simulink model "Plant"  (R2018b)
settings: configuration reference "plant_config" (kept outside this file)
values from neighbouring files (symbols this model uses):
  ada =     [acdata.mat]    (also in aero_data.mat)
  ade =     [acdata.mat]    (also in aero_data.mat)
  adr =     [acdata.mat]    (also in aero_data.mat)
  adyn =     [acdata.mat]    (also in aero_data.mat)
  alat =     [acdata.mat]    (also in aero_data.mat)
  alon =     [acdata.mat]    (also in aero_data.mat)
  geo =     [acdata.mat]    (also in aero_data.mat)
  mc =     [acdata.mat]    (also in aero_data.mat)
  PLANT_EXPORT = Simulink.Parameter(PLANT_EXPORT_VALUE)    [plant_model_init.m]
undefined symbols (not defined in the file or in its folder): acc_x, acc_x_O, acc_y, acc_y_O, acc_z, acc_z_O, alt, alt_0, day, diff_pressure, DiscIntNeverNeededParam, fixType, flags, gSpeed, gyr_x, gyr_y, gyr_z, h_R, hAcc, heading, headingAcc, height, hMSL, hour, iTOW, lat, lon, M_BO, M_OB, mag_x, mag_y, mag_z, month, nano, numSV, pDOP, phi, PLANT_CONST, plant_model, pressure, psi, quat, reserved1, reserved2, rot_x_B, rot_y_B, rot_z_B, sAcc, sec, Sensor_Model, tAcc, temperature, temprature, theta, timestamp, Va, vAcc, valid, vel_x_O, vel_y_O ... (+7)
libraries: FMT_Model_Lib x22, simulink x13, dspsrcs4 x6, aerolibatmos2 x1
(part 2 of 3)

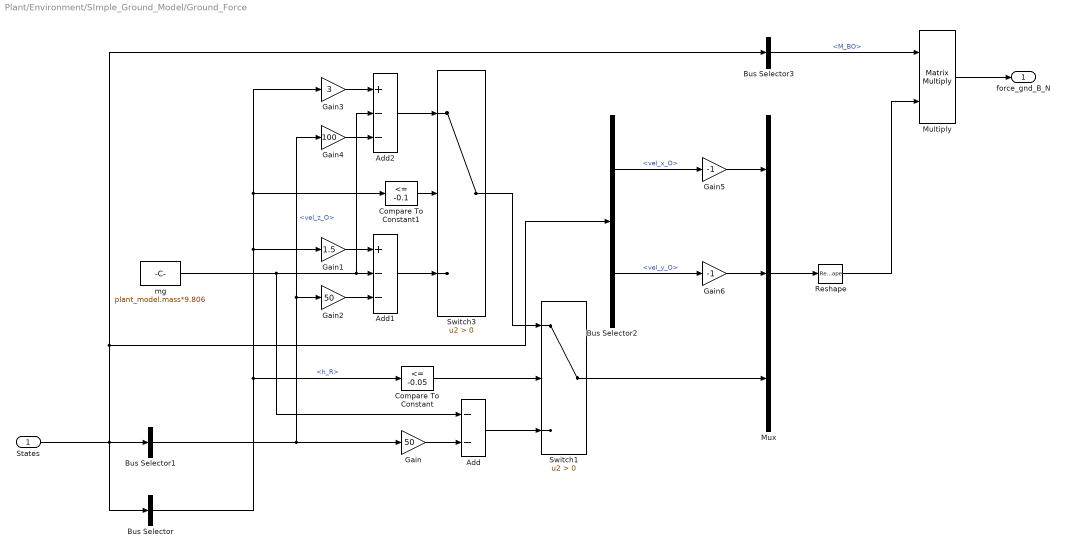
== system Plant/Environment/SImple_Ground_Model/Ground_Force ==
  States : Inport
  Add : Sum  Inputs=--
  Add1 : Sum  Inputs=+--
  Add2 : Sum  Inputs=+--
  Bus Selector : BusSelector  OutputSignals=Plant_States.h_R
  Bus Selector1 : BusSelector  OutputSignals=Plant_States.vel_z_O
  Bus Selector2 : BusSelector  OutputSignals=Plant_States.vel_x_O,Plant_States.vel_y_O
  Bus Selector3 : BusSelector  OutputSignals=Extended_States.M_BO
  Compare To Constant : simulink/Logic and Bit Operations/Compare To Constant  relop=<=  const=-0.05  OutDataTypeStr=boolean
  Compare To Constant1 : simulink/Logic and Bit Operations/Compare To Constant  relop=<=  const=-0.1  OutDataTypeStr=boolean
  Gain : Gain  Gain=50
  Gain1 : Gain  Gain=1.5
  Gain2 : Gain  Gain=50
  Gain3 : Gain  Gain=3
  Gain4 : Gain  Gain=100
  Gain5 : Gain  Gain=-1
  Gain6 : Gain  Gain=-1
  Multiply : Product  Multiplication=Matrix(*)
  Mux : Mux  Inputs=3
  Reshape : Reshape  OutputDimensionality=Customize  OutputDimensions=[3,1]
  Switch1 : Switch  Criteria=u2 > Threshold
  Switch3 : Switch  Criteria=u2 > Threshold
  mg : Constant  Value=plant_model.mass*9.806  OutDataTypeStr=single
  force_gnd_B_N : Outport
  wires:
  Switch1/1 -> Mux/3
  Bus Selector/1 -> Compare To Constant/1, Gain1/1, Gain3/1, Compare To Constant1/1  "<h_R>"
  Bus Selector1/1 -> Gain4/1, Gain2/1, Gain/1  "<vel_z_O>"
  Switch3/1 -> Switch1/1
  Gain1/1 -> Add1/1
  Gain5/1 -> Mux/1
  Gain3/1 -> Add2/1
  Compare To Constant/1 -> Switch1/2
  mg/1 -> Add/1, Add2/2, Add1/2
  Gain/1 -> Add/2
  Bus Selector2/2 -> Gain6/1  "<vel_y_O>"
  Gain2/1 -> Add1/3
  Add/1 -> Switch1/3
  Add2/1 -> Switch3/1
  Bus Selector2/1 -> Gain5/1  "<vel_x_O>"
  Gain6/1 -> Mux/2
  Compare To Constant1/1 -> Switch3/2
  Gain4/1 -> Add2/3
  Add1/1 -> Switch3/3
  Bus Selector3/1 -> Multiply/1  "<M_BO>"
  Mux/1 -> Reshape/1
  Multiply/1 -> force_gnd_B_N/1
  Reshape/1 -> Multiply/2
  States/1 -> Bus Selector/1, Bus Selector1/1, Bus Selector3/1, Bus Selector2/1

== system Plant/Environment/SImple_Ground_Model/Ground_Torque ==
  States : Inport
  Bus Selector2 : BusSelector  OutputSignals=Plant_States.rot_x_B,Plant_States.rot_y_B,Plant_States.rot_z_B
  Bus Selector3 : BusSelector  OutputSignals=Plant_States.phi,Plant_States.theta
  Constant : Constant  Value=0  OutDataTypeStr=single
  Gain1 : Gain  Gain=5
  Gain2 : Gain  Gain=plant_model.mass*9.806/30
  Gain3 : Gain  Gain=30
  Mux : Mux  Inputs=3
  Mux1 : Mux  Inputs=3
  Reshape1 : Reshape  OutputDimensionality=Customize  OutputDimensions=[3,1]
  Subtract : Sum  Inputs=--
  torque_gnd_B_Nm : Outport
  wires:
  Reshape1/1 -> Gain2/1
  States/1 -> Bus Selector3/1, Bus Selector2/1
  Subtract/1 -> Reshape1/1
  Bus Selector2/1 -> Mux1/1  "<rot_x_B>"
  Bus Selector2/2 -> Mux1/2  "<rot_y_B>"
  Bus Selector2/3 -> Mux1/3  "<rot_z_B>"
  Mux1/1 -> Gain1/1
  Gain1/1 -> Subtract/2
  Constant/1 -> Mux/3
  Mux/1 -> Gain3/1
  Gain2/1 -> torque_gnd_B_Nm/1
  Gain3/1 -> Subtract/1
  Bus Selector3/1 -> Mux/1  "<phi>"
  Bus Selector3/2 -> Mux/2  "<theta>"

== system Plant/Kinematic_Equation/Attitude_Dynamic/Quaternuin_Update ==
  omega_B_radPs : Inport
  reset : Inport  Port=2
  init_quat : Inport  Port=3
  Discrete-Time Integrator : DiscreteIntegrator  ExternalReset=level  InitialConditionSource=external  SampleTime=-1  ICPrevOutput=DiscIntNeverNeededParam  ICPrevScaledInput=DiscIntNeverNeededParam
  Gain : Gain  Gain=0.5  OutDataTypeStr=Inherit: Same as input
  Multiply : Product  Multiplication=Matrix(*)  OutDataTypeStr=Inherit: Same as first input
  Quaternion_Update_Maxtrix : Subsystem
  quat : Outport
  wires:
  Gain/1 -> Discrete-Time Integrator/1  "dot_q"
  Discrete-Time Integrator/1 -> quat/1, Multiply/2
  init_quat/1 -> Discrete-Time Integrator/3
  reset/1 -> Discrete-Time Integrator/2
  Multiply/1 -> Gain/1
  Quaternion_Update_Maxtrix/1(W) -> Multiply/1
  omega_B_radPs/1 -> Quaternion_Update_Maxtrix/1(omega_B_radPs)

== system Plant/Sensor_Model/Sensor_Airspeed/Airspeed ==
  Enable_Errors : Inport
  States : Inport  Port=2
  Bus Selector : BusSelector  OutputSignals=Extended_States.Va
  Gain : Gain  Gain=1.225/2
  Square : Math  Operator=square  SaturateOnIntegerOverflow=on
  Terminator : Terminator
  diff_pressure_Pa : Outport
  wires:
  States/1 -> Bus Selector/1
  Gain/1 -> diff_pressure_Pa/1
  Enable_Errors/1 -> Terminator/1
  Bus Selector/1 -> Square/1  "<Va>"
  Square/1 -> Gain/1

== system Plant/Sensor_Model/Sensor_Airspeed/Bus_Constructor ==
  diff_pressure_Pa : Inport  Unit=N/m^2
  timestamp_ms : Inport  Port=2
  Bus Assignment : BusAssignment  AssignedSignals=timestamp,diff_pressure
  Constant : Constant  Value=0  OutDataTypeStr=Bus: AirSpeed_Bus
  Data Type Conversion : DataTypeConversion  OutDataTypeStr=single
  Rate Transition : RateTransition  OutPortSampleTime=0.004
  Airspeed_Bus : Outport
  wires:
  Constant/1 -> Bus Assignment/1
  Data Type Conversion/1 -> Bus Assignment/3
  Bus Assignment/1 -> Rate Transition/1
  diff_pressure_Pa/1 -> Data Type Conversion/1
  Rate Transition/1 -> Airspeed_Bus/1
  timestamp_ms/1 -> Bus Assignment/2

== system Plant/Sensor_Model/Sensor_Barometer/Barometer ==
  Enable_Errors : Inport
  States : Inport  Port=2
  Physical_Model : Subsystem
  Sensor_Model : Subsystem
  pressure_Pa : Outport
  temprature_K : Outport  Port=2
  wires:
  Physical_Model/1(Pressure_Pa) -> Sensor_Model/2(u)
  Enable_Errors/1 -> Sensor_Model/1(Enable_Errors)
  States/1 -> Physical_Model/1(States)
  Sensor_Model/1(y) -> pressure_Pa/1
  Physical_Model/2(Temperature_K) -> temprature_K/1

== system Plant/Sensor_Model/Sensor_Barometer/Bus_Constructor ==
  pressure_Pa : Inport  Unit=N/m^2
  temperature_K : Inport  Port=2  Unit=K
  timestamp_ms : Inport  Port=3
  Bus Assignment : BusAssignment  AssignedSignals=timestamp,pressure,temperature
  Constant : Constant  Value=0  OutDataTypeStr=Bus: Barometer_Bus
  Constant2 : Constant  Value=273.15
  Data Type Conversion : DataTypeConversion  OutDataTypeStr=single
  Data Type Conversion1 : DataTypeConversion  OutDataTypeStr=single
  Rate Transition : RateTransition  OutPortSampleTime=0.01
  Sum1 : Sum  Inputs=|+-
  Barometer_Bus : Outport
  wires:
  Data Type Conversion1/1 -> Bus Assignment/4
  Constant/1 -> Bus Assignment/1
  Data Type Conversion/1 -> Bus Assignment/3
  Bus Assignment/1 -> Rate Transition/1
  pressure_Pa/1 -> Data Type Conversion/1
  temperature_K/1 -> Sum1/1
  Rate Transition/1 -> Barometer_Bus/1
  Sum1/1 -> Data Type Conversion1/1
  Constant2/1 -> Sum1/2
  timestamp_ms/1 -> Bus Assignment/2

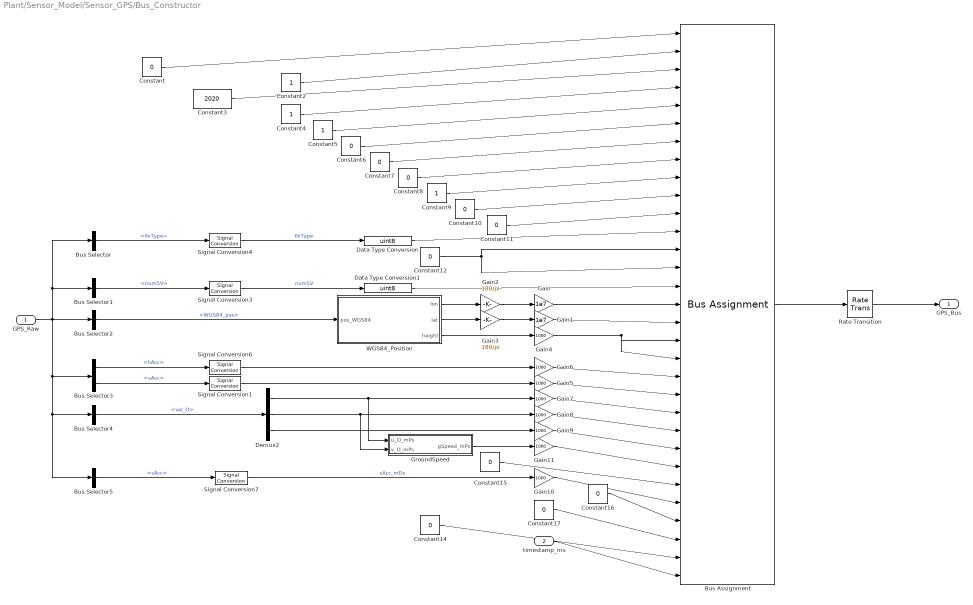
== system Plant/Sensor_Model/Sensor_GPS/Bus_Constructor ==
  GPS_Raw : Inport
  timestamp_ms : Inport  Port=2
  Bus Assignment : BusAssignment  AssignedSignals=iTOW,year,month,day,hour,min,sec,valid,tAcc,nano,fixType,flags,reserved1,numSV,lon,lat,height,hMSL,hAcc,vAcc,velN,velE,velD,gSpeed,heading,sAcc,headingAcc,pDOP,reserved2,timestamp
  Bus Selector : BusSelector  OutputSignals=fixType
  Bus Selector1 : BusSelector  OutputSignals=numSV
  Bus Selector2 : BusSelector  OutputSignals=WGS84_pos
  Bus Selector3 : BusSelector  OutputSignals=hAcc,vAcc
  Bus Selector4 : BusSelector  OutputSignals=vel_O
  Bus Selector5 : BusSelector  OutputSignals=sAcc
  Constant : Constant  Value=0  OutDataTypeStr=Bus: GPS_uBlox_Bus
  Constant10 : Constant  Value=0  OutDataTypeStr=uint32
  Constant11 : Constant  Value=0  OutDataTypeStr=int32
  Constant{6..8,12} (4 alike) : Constant  Value=0  OutDataTypeStr=uint8
  Constant14 : Constant  Value=0  OutDataTypeStr=uint16
  Constant15 : Constant  Value=0  OutDataTypeStr=int32
  Constant16 : Constant  Value=0  OutDataTypeStr=uint32
  Constant17 : Constant  Value=0  OutDataTypeStr=uint16
  Constant2 : Constant  OutDataTypeStr=uint32
  Constant3 : Constant  Value=2020  OutDataTypeStr=uint16
  Constant4 : Constant  OutDataTypeStr=uint8
  Constant5 : Constant  OutDataTypeStr=uint8
  Constant9 : Constant  OutDataTypeStr=uint8
  Data Type Conversion : DataTypeConversion  OutDataTypeStr=uint8
  Data Type Conversion1 : DataTypeConversion  OutDataTypeStr=uint8
  Demux2 : Demux  Outputs=3
  Gain : Gain  Gain=1e7  OutDataTypeStr=int32
      settings: AttributesFormatString=Gain: %<Gain>
  Gain1 : Gain  Gain=1e7  OutDataTypeStr=int32
      settings: AttributesFormatString=Gain: %<Gain>
  Gain10 : Gain  Gain=1000  OutDataTypeStr=uint32
      settings: AttributesFormatString=Gain: %<Gain>
  Gain{4,7..9,11} (5 alike) : Gain  Gain=1000  OutDataTypeStr=int32
      settings: AttributesFormatString=Gain: %<Gain>
  Gain2 : Gain  Gain=180/pi
      settings: AttributesFormatString=Gain: %<Gain>
  Gain3 : Gain  Gain=180/pi
      settings: AttributesFormatString=Gain: %<Gain>
  Gain5 : Gain  Gain=1000  OutDataTypeStr=uint32
      settings: AttributesFormatString=Gain: %<Gain>
  Gain6 : Gain  Gain=1000  OutDataTypeStr=uint32
      settings: AttributesFormatString=Gain: %<Gain>
  GroundSpeed : Subsystem
  Rate Transition : RateTransition  OutPortSampleTime=0.1
  Signal Conversion{1,3..4,6..7} (5 alike) : SignalConversion  OverrideOpt=off
  WGS84_Position : Subsystem
  GPS_Bus : Outport
  wires:
  Bus Selector5/1 -> Signal Conversion7/1  "<sAcc>"
  Bus Selector3/1 -> Signal Conversion6/1  "<hAcc>"
  Bus Selector1/1 -> Signal Conversion3/1  "<numSV>"
  Bus Selector4/1 -> Demux2/1  "<vel_O>"
  Gain5/1 -> Bus Assignment/21
  Constant15/1 -> Bus Assignment/26
  Data Type Conversion/1 -> Bus Assignment/12
  Constant17/1 -> Bus Assignment/29
  Gain4/1 -> Bus Assignment/19, Bus Assignment/18
  Constant16/1 -> Bus Assignment/28
  Gain3/1 -> Gain1/1
  Signal Conversion6/1 -> Gain6/1
  Gain6/1 -> Bus Assignment/20
  Gain11/1 -> Bus Assignment/25
  Gain8/1 -> Bus Assignment/23
  Gain7/1 -> Bus Assignment/22
  Gain10/1 -> Bus Assignment/27
  Constant/1 -> Bus Assignment/1
  Constant8/1 -> Bus Assignment/8
  Gain2/1 -> Gain/1
  Constant4/1 -> Bus Assignment/4
  Constant11/1 -> Bus Assignment/11
  Constant10/1 -> Bus Assignment/10
  Constant9/1 -> Bus Assignment/9
  Constant3/1 -> Bus Assignment/3
  Constant6/1 -> Bus Assignment/6
  Bus Assignment/1 -> Rate Transition/1
  Gain9/1 -> Bus Assignment/24
  Constant12/1 -> Bus Assignment/14, Bus Assignment/13
  Constant14/1 -> Bus Assignment/30
  GroundSpeed/1(gSpeed_mPs) -> Gain11/1
  Constant5/1 -> Bus Assignment/5
  Gain/1 -> Bus Assignment/16
  Data Type Conversion1/1 -> Bus Assignment/15
  Constant2/1 -> Bus Assignment/2
  Gain1/1 -> Bus Assignment/17
  Constant7/1 -> Bus Assignment/7
  Signal Conversion7/1 -> Gain10/1  "sAcc_mDs"
  Demux2/1 -> GroundSpeed/1(u_O_mPs), Gain7/1
  Demux2/2 -> Gain8/1, GroundSpeed/2(v_O_mPs)
  Demux2/3 -> Gain9/1
  Bus Selector2/1 -> WGS84_Position/1(pos_WGS84)  "<WGS84_pos>"
  WGS84_Position/1(lon) -> Gain2/1
  WGS84_Position/2(lat) -> Gain3/1
  WGS84_Position/3(height) -> Gain4/1
  Signal Conversion3/1 -> Data Type Conversion1/1  "numSV"
  Signal Conversion4/1 -> Data Type Conversion/1  "fixType"
  Bus Selector3/2 -> Signal Conversion1/1  "<vAcc>"
  Signal Conversion1/1 -> Gain5/1
  Rate Transition/1 -> GPS_Bus/1
  timestamp_ms/1 -> Bus Assignment/31
  GPS_Raw/1 -> Bus Selector3/1, Bus Selector4/1, Bus Selector5/1, Bus Selector2/1, Bus Selector1/1, Bus Selector/1
  Bus Selector/1 -> Signal Conversion4/1  "<fixType>"

== system Plant/Sensor_Model/Sensor_GPS/GPS ==
  Enable_Errors : Inport
  States : Inport  Port=2
  Bus_Constructor : Subsystem
  Physical_Model : Subsystem
  Sensor_Model : Subsystem
  GPS_Raw : Outport
  wires:
  Physical_Model/1(WGS84_pos_rad) -> Sensor_Model/2(WGS84_pos_rad)
  Physical_Model/2(vel_O_mPs) -> Sensor_Model/3(vel_O_mPs)
  States/1 -> Physical_Model/1(States)
  Enable_Errors/1 -> Sensor_Model/1(Enable_Errors)
  Sensor_Model/1(WGS84_pos_meas) -> Bus_Constructor/1(WGS84_pos_meas)
  Sensor_Model/2(vel_O_meas) -> Bus_Constructor/2(vel_O_meas)
  Sensor_Model/3(numSV) -> Bus_Constructor/3(numSV)
  Sensor_Model/4(fixType) -> Bus_Constructor/4(fixType)
  Sensor_Model/5(h_Acc_m) -> Bus_Constructor/5(h_Acc_m)
  Sensor_Model/6(v_Acc_m) -> Bus_Constructor/6(v_Acc_m)
  Sensor_Model/7(s_Acc_mDs) -> Bus_Constructor/7(s_Acc_mDs)
  Bus_Constructor/1(GPS_Raw) -> GPS_Raw/1

== system Plant/Sensor_Model/Sensor_IMU/Accelerometer ==
  States : Inport
  Enable_Errors : Inport  Port=2
  Bus_Constructor : Subsystem
  Physical_Model : Subsystem
  Sensor_Model : Subsystem
  Acc_Raw : Outport
  wires:
  Sensor_Model/1(y) -> Bus_Constructor/1(Output)
  States/1 -> Physical_Model/1(States)
  Physical_Model/1(sfor_B_mPs2) -> Sensor_Model/2(u)
  Bus_Constructor/1(Acc_Raw) -> Acc_Raw/1
  Enable_Errors/1 -> Physical_Model/2(Enable_Errors), Sensor_Model/1(Enable_Errors)

== system Plant/Sensor_Model/Sensor_IMU/Bus_Constructor ==
  Gyro_Raw : Inport
  Acc_Raw : Inport  Port=2
  timestamp_ms : Inport  Port=3
  Bus Assignment : BusAssignment  AssignedSignals=timestamp,gyr_x,gyr_y,gyr_z,acc_x,acc_y,acc_z
  Bus Selector : BusSelector  OutputSignals=Gyro_x_radPs,Gyro_y_radPs,Gyro_z_radPs
  Bus Selector1 : BusSelector  OutputSignals=Acc_x_mPs2,Acc_y_mPs2,Acc_z_mPs2
  Constant : Constant  Value=0  OutDataTypeStr=Bus: IMU_Bus
  IMU_Bus : Outport
  wires:
  Gyro_Raw/1 -> Bus Selector/1
  Acc_Raw/1 -> Bus Selector1/1
  Constant/1 -> Bus Assignment/1
  timestamp_ms/1 -> Bus Assignment/2
  Bus Assignment/1 -> IMU_Bus/1
  Bus Selector/1 -> Bus Assignment/3  "<Gyro_x_radPs>"
  Bus Selector/2 -> Bus Assignment/4  "<Gyro_y_radPs>"
  Bus Selector/3 -> Bus Assignment/5  "<Gyro_z_radPs>"
  Bus Selector1/1 -> Bus Assignment/6  "<Acc_x_mPs2>"
  Bus Selector1/2 -> Bus Assignment/7  "<Acc_y_mPs2>"
  Bus Selector1/3 -> Bus Assignment/8  "<Acc_z_mPs2>"

== system Plant/Sensor_Model/Sensor_IMU/Gyroscope ==
  States : Inport
  Enable_Errors : Inport  Port=2
  Bus_Constructor : Subsystem
  Physical_Model : Subsystem
  Sensor_Model : Subsystem
  Gyro_Raw : Outport
  wires:
  States/1 -> Physical_Model/1(States)
  Sensor_Model/1(y) -> Bus_Constructor/1(Output)
  Bus_Constructor/1(Gyro_Raw) -> Gyro_Raw/1
  Enable_Errors/1 -> Physical_Model/2(Enable_Errors), Sensor_Model/1(Enable_Errors)
  Physical_Model/1(gyr_B_radDs) -> Sensor_Model/2(u)

== system Plant/Sensor_Model/Sensor_MAG/Bus_Constructor ==
  Mag_Raw : Inport
  timestamp_ms : Inport  Port=2
  Bus Assignment : BusAssignment  AssignedSignals=timestamp,mag_x,mag_y,mag_z
  Bus Selector : BusSelector  OutputSignals=Mag_x_gauss,Mag_y_gauss,Mag_z_gauss
  Constant : Constant  Value=0  OutDataTypeStr=Bus: MAG_Bus
  Rate Transition : RateTransition  OutPortSampleTime=0.01
  MAG_Bus : Outport
  wires:
  Bus Assignment/1 -> Rate Transition/1
  Constant/1 -> Bus Assignment/1
  timestamp_ms/1 -> Bus Assignment/2
  Rate Transition/1 -> MAG_Bus/1
  Bus Selector/1 -> Bus Assignment/3  "<Mag_x_gauss>"
  Mag_Raw/1 -> Bus Selector/1
  Bus Selector/2 -> Bus Assignment/4  "<Mag_y_gauss>"
  Bus Selector/3 -> Bus Assignment/5  "<Mag_z_gauss>"

== system Plant/Sensor_Model/Sensor_MAG/Magnetometer ==
  States : Inport
  Enable_Errors : Inport  Port=2
  Bus_Constructor : Subsystem
  Physical_Model : Subsystem
  Sensor_Model : Subsystem
  Mag_Raw : Outport
  wires:
  Bus_Constructor/1(Mag_Raw) -> Mag_Raw/1
  Sensor_Model/1(y) -> Bus_Constructor/1(Output)
  States/1 -> Physical_Model/1(States)
  Physical_Model/1(mag_B_gauss) -> Sensor_Model/2(u)
  Enable_Errors/1 -> Sensor_Model/1(Enable_Errors)

== system Plant/Actuators/Aerodynamics Forces and Moments/Actuator Command/aileron_cmd ==
  actuator_cmd : Inport
  Bias : Bias  Bias=-1500
  Data Type Conversion : DataTypeConversion  OutDataTypeStr=single
  Gain2 : Gain  Gain=(30/500)*(pi/180)
  Selector : Selector  InputPortWidth=16  IndexOptions=Index vector (dialog)  Indices=6  OutputSizes=1
  aileron_cmd : Outport
  wires:
  actuator_cmd/1 -> Selector/1
  Gain2/1 -> aileron_cmd/1
  Bias/1 -> Gain2/1
  Selector/1 -> Data Type Conversion/1
  Data Type Conversion/1 -> Bias/1

== system Plant/Actuators/Aerodynamics Forces and Moments/Actuator Command/elevator_cmd ==
  actuator_cmd : Inport
  Bias : Bias  Bias=-1500
  Data Type Conversion : DataTypeConversion  OutDataTypeStr=single
  Gain2 : Gain  Gain=(30/500)*(pi/180)
  Selector : Selector  InputPortWidth=16  IndexOptions=Index vector (dialog)  Indices=8  OutputSizes=1
  elevator_cmd : Outport
  wires:
  Data Type Conversion/1 -> Bias/1
  Selector/1 -> Data Type Conversion/1
  Bias/1 -> Gain2/1
  Gain2/1 -> elevator_cmd/1
  actuator_cmd/1 -> Selector/1

== system Plant/Actuators/Aerodynamics Forces and Moments/Actuator Command/rudder_cmd ==
  actuator_cmd : Inport
  Bias : Bias  Bias=-1500
  Data Type Conversion : DataTypeConversion  OutDataTypeStr=single
  Gain2 : Gain  Gain=(30/500)*(pi/180)
  Selector : Selector  InputPortWidth=16  IndexOptions=Index vector (dialog)  Indices=9  OutputSizes=1
  rudder_cmd : Outport
  wires:
  Data Type Conversion/1 -> Bias/1
  Selector/1 -> Data Type Conversion/1
  Bias/1 -> Gain2/1
  Gain2/1 -> rudder_cmd/1
  actuator_cmd/1 -> Selector/1

== system Plant/Actuators/Aerodynamics Forces and Moments/Aerodynamic Coefficients/Actuator increments ==
  Incid : Inport
  ActData : Inport  Port=2
  Demux : Demux  Outputs=2
  Demux1 : Demux  Outputs=3
  Sum1 : Sum  Inputs=|+++
  Terminator : Terminator
  aileron : Subsystem
  elevator : Subsystem
  rudder : Subsystem
  Coeffs : Outport
  wires:
  Demux/2 -> Terminator/1
  Incid/1 -> Demux/1
  Demux/1 -> rudder/1(alpha), elevator/1(alpha), aileron/1(alpha)
  ActData/1 -> Demux1/1
  elevator/1(Coeffs) -> Sum1/2
  Sum1/1 -> Coeffs/1
  rudder/1(Coeffs) -> Sum1/3
  aileron/1(Coeffs) -> Sum1/1
  Demux1/3 -> rudder/2(dr)
  Demux1/2 -> elevator/2(de)
  Demux1/1 -> aileron/2(da)

== system Plant/Actuators/Aerodynamics Forces and Moments/Aerodynamic Coefficients/Basic Coefficients ==
  incid : Inport
  CD_basic : Lookup  InputValues=alon.alpha  Table=alon.CD
  CD_beta : Lookup2D  RowIndex=alat.beta  ColumnIndex=alat.alpha  Table=alat.CD
  CL_basic : Lookup  InputValues=alon.alpha  Table=alon.CL
  CL_beta : Lookup2D  RowIndex=alat.beta  ColumnIndex=alat.alpha  Table=alat.CL
  CY_basic : Lookup2D  RowIndex=alat.beta  ColumnIndex=alat.alpha  Table=alat.CY
  Cl_basic : Lookup2D  RowIndex=alat.beta  ColumnIndex=alat.alpha  Table=alat.Cl
  Cm_basic : Lookup  InputValues=alon.alpha  Table=alon.Cm
  Cm_beta : Lookup2D  RowIndex=alat.beta  ColumnIndex=alat.alpha  Table=alat.Cm
  Cn_basic : Lookup2D  RowIndex=alat.beta  ColumnIndex=alat.alpha  Table=alat.Cn  LookUpMeth=Interpolation-Use End Values
  Demux : Demux  Outputs=2
  Mux : Mux  Inputs=6
  Sum : Sum  Inputs=|++
  Sum1 : Sum  Inputs=|++
  Sum2 : Sum  Inputs=|++
  Coeffs : Outport
  wires:
  incid/1 -> Demux/1
  Demux/1 -> CY_basic/2, Cl_basic/2, Cm_basic/1, Cn_basic/2, CL_beta/2, CD_beta/2, Cm_beta/2, CL_basic/1, CD_basic/1
  CL_basic/1 -> Sum/1
  CD_basic/1 -> Sum1/1
  Cm_basic/1 -> Sum2/1
  Sum/1 -> Mux/2  "CL"
  Sum1/1 -> Mux/1  "CD"
  Sum2/1 -> Mux/5  "Cm"
  Mux/1 -> Coeffs/1
  CL_beta/1 -> Sum/2
  CD_beta/1 -> Sum1/2
  Cm_beta/1 -> Sum2/2
  CY_basic/1 -> Mux/3  "CY"
  Cl_basic/1 -> Mux/4  "Cl"
  Cn_basic/1 -> Mux/6  "Cn"
  Demux/2 -> CY_basic/1, Cl_basic/1, Cn_basic/1, CL_beta/1, CD_beta/1, Cm_beta/1

== system Plant/Actuators/Aerodynamics Forces and Moments/Aerodynamic Coefficients/Coeff_Decay ==
  u : Inport
  Va : Inport  Port=2
  Abs : Abs
  Constant : Constant  Value=10
  Divide : Product  Inputs=*/
  Multiply : Product
  Square : Math  Operator=square  SaturateOnIntegerOverflow=on
  Switch : Switch  Threshold=10
  y : Outport
  wires:
  Switch/1 -> y/1
  Divide/1 -> Square/1
  Constant/1 -> Divide/2
  u/1 -> Multiply/1, Switch/1
  Multiply/1 -> Switch/3  "dd1"
  Va/1 -> Abs/1
  Abs/1 -> Switch/2, Divide/1
  Square/1 -> Multiply/2

== system Plant/Actuators/Aerodynamics Forces and Moments/Aerodynamic Coefficients/body axis forces ==
  Incid : Inport
  Cl_DLY : Inport  Port=2
  Cl_xA : Fcn  Expr=-u[3]*cos(u[2])*cos(u[1])+u[4]*sin(u[1])
  Cl_yA : Fcn  Expr=-u[3]*sin(u[2])+u[5]
  Cl_zA : Fcn  Expr=-u[3]*cos(u[2])*sin(u[1])-u[4]*cos(u[1])
  Mux : Mux  Inputs=3
  Mux1 : Mux  Inputs=2
  Cl_XYZ : Outport
  wires:
  Mux/1 -> Cl_XYZ/1
  Cl_DLY/1 -> Mux1/2
  Incid/1 -> Mux1/1
  Cl_zA/1 -> Mux/3
  Cl_yA/1 -> Mux/2
  Cl_xA/1 -> Mux/1
  Mux1/1 -> Cl_zA/1, Cl_yA/1, Cl_xA/1

== system Plant/Actuators/Aerodynamics Forces and Moments/Aerodynamic Coefficients/body rate damping ==
  Incid : Inport
  pqr_n : Inport  Port=2
  Add : Sum  Inputs=+++
  Demux : Demux  Outputs=2
  Demux1 : Demux  Outputs=3
  Saturation : Saturate  UpperLimit=15/180*pi  LowerLimit=-15/180*pi
  Terminator : Terminator
  p : Subsystem
  p1 : Product  RndMeth=Zero
  q : Subsystem
  q1 : Product  RndMeth=Zero
  r : Subsystem
  r1 : Product  RndMeth=Zero
  Coeffs : Outport
  wires:
  Incid/1 -> Demux/1
  Demux/1 -> Saturation/1
  Demux/2 -> Terminator/1
  pqr_n/1 -> Demux1/1
  p/1(Coeffs) -> p1/1
  Demux1/1 -> p1/2
  q/1(Coeffs) -> q1/1
  r/1(Coeffs) -> r1/1
  Demux1/2 -> q1/2
  Demux1/3 -> r1/2
  q1/1 -> Add/2
  p1/1 -> Add/1
  r1/1 -> Add/3
  Add/1 -> Coeffs/1
  Saturation/1 -> p/1(alpha), q/1(alpha), r/1(alpha)

== system Plant/Actuators/Aerodynamics Forces and Moments/Aerodynamic Forces and Moments/Moments about CG due to Forces ==
  Forces : Inport
  CG : Inport  Port=2
  CP : Inport  Port=3
  Cross Product : FMT_Model_Lib/Math/Cross Product
      settings: SourceProductName=FMT Toolbox
  Sum : Sum  Inputs=|+-
  Moments : Outport
  wires:
  Cross Product/1 -> Moments/1
  Sum/1 -> Cross Product/2
  Forces/1 -> Cross Product/1
  CG/1 -> Sum/1
  CP/1 -> Sum/2

== system Plant/Actuators/MainMotor Forces and Moments/ESCs/Rotor_Delay ==
  in : Inport
  Discrete-Time Integrator : DiscreteIntegrator  gainval=K  SampleTime=-1  ICPrevOutput=DiscIntNeverNeededParam  ICPrevScaledInput=DiscIntNeverNeededParam
  Gain : Gain  Gain=1/T
  Subtract : Sum  Inputs=+-
  out : Outport
  wires:
  in/1 -> Subtract/1
  Subtract/1 -> Gain/1
  Gain/1 -> Discrete-Time Integrator/1
  Discrete-Time Integrator/1 -> Subtract/2, out/1

== system Plant/Actuators/MainMotor Forces and Moments/ESCs/Rotor_Speed ==
  u0 : Inport
  Add : Sum
  Compare To Constant : simulink/Logic and Bit Operations/Compare To Constant  relop=>  const=0.1  OutDataTypeStr=boolean
  Constant1 : Constant  Value=p  OutDataTypeStr=single
  Gain1 : Gain  Gain=k  OutDataTypeStr=Inherit: Same as input
  Multiply : Product
  Saturation1 : Saturate  UpperLimit=9999999  LowerLimit=0
  omega_B_radPs : Outport
  wires:
  Multiply/1 -> Saturation1/1
  Gain1/1 -> Add/1
  Saturation1/1 -> omega_B_radPs/1
  u0/1 -> Compare To Constant/1, Gain1/1
  Constant1/1 -> Add/2
  Compare To Constant/1 -> Multiply/1
  Add/1 -> Multiply/2

== system Plant/Actuators/MainMotor Forces and Moments/Force/Rotor_Thrust ==
  rotor_speed_radPs : Inport
  Multiply : Product  OutDataTypeStr=Inherit: Same as first input
  Square : Math  Operator=square  SaturateOnIntegerOverflow=on
  cT : Constant  Value=cT
  thrust_B_N : Outport
  wires:
  rotor_speed_radPs/1 -> Square/1
  Square/1 -> Multiply/1
  cT/1 -> Multiply/2
  Multiply/1 -> thrust_B_N/1

== system Plant/Actuators/Motors Forces and Moments/ESCs/Rotor_Delay ==
  in : Inport
  Discrete-Time Integrator : DiscreteIntegrator  gainval=K  SampleTime=-1  ICPrevOutput=DiscIntNeverNeededParam  ICPrevScaledInput=DiscIntNeverNeededParam
  Gain : Gain  Gain=1/T
  Subtract : Sum  Inputs=+-
  out : Outport
  wires:
  in/1 -> Subtract/1
  Subtract/1 -> Gain/1
  Gain/1 -> Discrete-Time Integrator/1
  Discrete-Time Integrator/1 -> Subtract/2, out/1

== system Plant/Actuators/Motors Forces and Moments/ESCs/Rotor_Speed ==
  u0 : Inport
  Add : Sum
  Compare To Constant : simulink/Logic and Bit Operations/Compare To Constant  relop=>  const=0.1  OutDataTypeStr=boolean
  Constant1 : Constant  Value=p  OutDataTypeStr=single
  Gain1 : Gain  Gain=k  OutDataTypeStr=Inherit: Same as input
  Multiply : Product
  Saturation1 : Saturate  UpperLimit=9999999  LowerLimit=0
  omega_B_radPs : Outport
  wires:
  Multiply/1 -> Saturation1/1
  Gain1/1 -> Add/1
  Saturation1/1 -> omega_B_radPs/1
  u0/1 -> Compare To Constant/1, Gain1/1
  Constant1/1 -> Add/2
  Compare To Constant/1 -> Multiply/1
  Add/1 -> Multiply/2

== system Plant/Actuators/Motors Forces and Moments/Force/Rotor_Thrust ==
  rotor_speed_radPs : Inport
  Multiply : Product  OutDataTypeStr=Inherit: Same as first input
  Square : Math  Operator=square  SaturateOnIntegerOverflow=on
  cT : Constant  Value=cT
  thrust_B_N : Outport
  wires:
  rotor_speed_radPs/1 -> Square/1
  Square/1 -> Multiply/1
  cT/1 -> Multiply/2
  Multiply/1 -> thrust_B_N/1

== system Plant/Actuators/Motors Forces and Moments/Torque/Gyroscopic_Torque ==
  rotor_speed_radPs : Inport
  omega_B_radPs : Inport  Port=2
  Add : Sum  Inputs=--++
  Constant : Constant  Value=[0;0;Im]  OutDataTypeStr=single
  Cross Product : FMT_Model_Lib/Math/Cross Product
      settings: SourceProductName=FMT Toolbox
  Demux : Demux
  Multiply : Product
  gyroscopic_torque : Outport
  wires:
  Demux/1 -> Add/1
  Constant/1 -> Cross Product/1
  Demux/4 -> Add/4
  Add/1 -> Multiply/1
  Demux/3 -> Add/3
  Demux/2 -> Add/2
  omega_B_radPs/1 -> Multiply/2
  Multiply/1 -> Cross Product/2
  Cross Product/1 -> gyroscopic_torque/1
  rotor_speed_radPs/1 -> Demux/1

== system Plant/Actuators/Motors Forces and Moments/Torque/Rotor_Torque ==
  rotor_speed_radPs : Inport
  Multiply : Product  Multiplication=Matrix(*)
  Square : Math  Operator=square  SaturateOnIntegerOverflow=on
  X_Frame_CM : Constant  Value=[-L*cT,L*cT,L*cT,-L*cT;L*cT,-L*cT,L*cT,-L*cT;cQ,cQ,-cQ,-cQ]  OutDataTypeStr=single
  rotor_torque : Outport
  wires:
  X_Frame_CM/1 -> Multiply/1
  Square/1 -> Multiply/2
  Multiply/1 -> rotor_torque/1
  rotor_speed_radPs/1 -> Square/1

== system Plant/Kinematic_Equation/Attitude_Dynamic/Quaternuin_Update/Quaternion_Update_Maxtrix ==
  omega_B_radPs : Inport
  Constant{,1..3} (4 alike) : Constant  Value=0  OutDataTypeStr=single
  Demux : Demux  Outputs=3
  Gain{1..4,6..7} (6 alike) : Gain  Gain=-1  OutDataTypeStr=Inherit: Same as input
  Matrix Concatenate{,1..3} (4 alike) : Concatenate  NumInputs=4
  Matrix Concatenate4 : Concatenate  NumInputs=4  Mode=Multidimensional array  ConcatenateDimension=2
  W : Outport
  wires:
  Gain1/1 -> Matrix Concatenate1/1
  Gain7/1 -> Matrix Concatenate3/2
  Matrix Concatenate2/1 -> Matrix Concatenate4/3  "col3"
  Constant2/1 -> Matrix Concatenate2/3
  Matrix Concatenate4/1 -> W/1
  Demux/1 -> Matrix Concatenate/2, Gain1/1, Gain4/1, Matrix Concatenate3/3  "w1"
  Matrix Concatenate/1 -> Matrix Concatenate4/1  "col1"
  Matrix Concatenate1/1 -> Matrix Concatenate4/2  "col2"
  Constant3/1 -> Matrix Concatenate3/4
  Gain6/1 -> Matrix Concatenate3/1
  Constant1/1 -> Matrix Concatenate1/2
  Matrix Concatenate3/1 -> Matrix Concatenate4/4  "col4"
  Demux/2 -> Matrix Concatenate1/4, Gain3/1, Gain7/1, Matrix Concatenate/3  "w2"
  Constant/1 -> Matrix Concatenate/1
  Gain3/1 -> Matrix Concatenate2/1
  Demux/3 -> Gain2/1, Matrix Concatenate2/2, Gain6/1, Matrix Concatenate/4  "w3"
  Gain2/1 -> Matrix Concatenate1/3
  omega_B_radPs/1 -> Demux/1
  Gain4/1 -> Matrix Concatenate2/4

== system Plant/Sensor_Model/Sensor_Barometer/Barometer/Physical_Model ==
  States : Inport
  Bus Selector1 : BusSelector  OutputSignals=Plant_States.alt
  Data Type Conversion : DataTypeConversion  OutDataTypeStr=single
  ISA Atmosphere Model : aerolibatmos2/ISA Atmosphere Model  custom=off  g=9.80665  gamma=1.4  R=287.0531  L=0.0065  h_trop=11000  h_strat=20000  rho0=1.225  P0=101325  T0=288.15  h0=0
      settings: SourceProductName=Aerospace Blockset
  Terminator : Terminator
  Terminator1 : Terminator
  Pressure_Pa : Outport
  Temperature_K : Outport  Port=2
  wires:
  States/1 -> Bus Selector1/1
  ISA Atmosphere Model/1 -> Temperature_K/1
  ISA Atmosphere Model/2 -> Terminator1/1
  ISA Atmosphere Model/4 -> Terminator/1
  Bus Selector1/1 -> Data Type Conversion/1  "<alt>"
  ISA Atmosphere Model/3 -> Pressure_Pa/1
  Data Type Conversion/1 -> ISA Atmosphere Model/1

== system Plant/Sensor_Model/Sensor_Barometer/Barometer/Sensor_Model ==
  Enable_Errors : Inport
  u : Inport  Port=2
  Add : Sum  InputSameDT=on  OutDataTypeStr=Inherit: Same as first input
  Saturation : Saturate  UpperLimit=Sensor_Model.Baro.Upper_limit  LowerLimit=Sensor_Model.Baro.Lower_limit  OutDataTypeStr=single
  Sensor_Error : Subsystem
  Sensor_Noise : Subsystem
  Switch : Switch  Criteria=u2 > Threshold
  y : Outport
  wires:
  Switch/1 -> y/1
  Saturation/1 -> Add/1
  Sensor_Error/1(y) -> Saturation/1
  Enable_Errors/1 -> Switch/2
  u/1 -> Switch/3, Sensor_Error/1(u)
  Add/1 -> Switch/1
  Sensor_Noise/1(noise) -> Add/2

== system Plant/Sensor_Model/Sensor_GPS/Bus_Constructor/GroundSpeed ==
  u_O_mPs : Inport
  v_O_mPs : Inport  Port=2
  Add : Sum
  Math Function : Math  Operator=square  SaturateOnIntegerOverflow=on
  Math Function1 : Math  Operator=square  SaturateOnIntegerOverflow=on
  Saturation : Saturate  UpperLimit=inf  LowerLimit=0
  Sqrt : Sqrt  SaturateOnIntegerOverflow=on
  gSpeed_mPs : Outport
  wires:
  Sqrt/1 -> gSpeed_mPs/1
  Math Function/1 -> Add/1
  Math Function1/1 -> Add/2
  Saturation/1 -> Sqrt/1
  Add/1 -> Saturation/1
  u_O_mPs/1 -> Math Function/1
  v_O_mPs/1 -> Math Function1/1

== system Plant/Sensor_Model/Sensor_GPS/Bus_Constructor/WGS84_Position ==
  pos_WGS84 : Inport
  Demux1 : Demux  Outputs=3
  Signal Conversion : SignalConversion  OverrideOpt=off
  Signal Conversion1 : SignalConversion  OverrideOpt=off
  Signal Conversion2 : SignalConversion  OverrideOpt=off
  lon : Outport
  lat : Outport  Port=2
  height : Outport  Port=3
  wires:
  Demux1/3 -> Signal Conversion2/1  "POS_h_WGS84"
  Signal Conversion/1 -> lon/1
  Demux1/1 -> Signal Conversion/1  "POS_lon_WGS84"
  pos_WGS84/1 -> Demux1/1
  Demux1/2 -> Signal Conversion1/1  "POS_lat_WGS84"
  Signal Conversion1/1 -> lat/1
  Signal Conversion2/1 -> height/1

== system Plant/Sensor_Model/Sensor_GPS/GPS/Bus_Constructor ==
  WGS84_pos_meas : Inport
  vel_O_meas : Inport  Port=2
  numSV : Inport  Port=3
  fixType : Inport  Port=4
  h_Acc_m : Inport  Port=5
  v_Acc_m : Inport  Port=6
  s_Acc_mDs : Inport  Port=7
  Bus Creator : BusCreator  Inputs=7
  GPS_Raw : Outport
  wires:
  WGS84_pos_meas/1 -> Bus Creator/1  "WGS84_pos"
  vel_O_meas/1 -> Bus Creator/2  "vel_O"
  numSV/1 -> Bus Creator/3  "numSV"
  fixType/1 -> Bus Creator/4  "fixType"
  h_Acc_m/1 -> Bus Creator/5  "hAcc"
  v_Acc_m/1 -> Bus Creator/6  "vAcc"
  s_Acc_mDs/1 -> Bus Creator/7  "sAcc"
  Bus Creator/1 -> GPS_Raw/1

== system Plant/Sensor_Model/Sensor_GPS/GPS/Physical_Model ==
  note: Transfer Delay
  States : Inport
  Bus Selector : BusSelector  OutputSignals=Plant_States.lon,Plant_States.lat,Plant_States.alt
  Bus Selector1 : BusSelector  OutputSignals=Plant_States.vel_x_O,Plant_States.vel_y_O,Plant_States.vel_z_O
  Delay : Delay  DelayLength=150/(PLANT_CONST.dt*1e3)
  Delay1 : Delay  DelayLength=100/(PLANT_CONST.dt*1e3)
  Vector Concatenate : Concatenate  NumInputs=3  Mode=Multidimensional array
  Vector Concatenate1 : Concatenate  NumInputs=3  Mode=Multidimensional array
  WGS84_pos_rad : Outport  Unit=rad/s
  vel_O_mPs : Outport  Port=2  Unit=m/s  PortDimensions=[3 1]
  wires:
  Bus Selector/3 -> Vector Concatenate/3  "<alt>"
  Bus Selector/2 -> Vector Concatenate/2  "<lat>"
  Bus Selector/1 -> Vector Concatenate/1  "<lon>"
  Vector Concatenate/1 -> Delay/1
  Bus Selector1/2 -> Vector Concatenate1/2  "<vel_y_O>"
  Bus Selector1/3 -> Vector Concatenate1/3  "<vel_z_O>"
  States/1 -> Bus Selector1/1, Bus Selector/1
  Vector Concatenate1/1 -> Delay1/1
  Bus Selector1/1 -> Vector Concatenate1/1  "<vel_x_O>"
  Delay/1 -> WGS84_pos_rad/1
  Delay1/1 -> vel_O_mPs/1

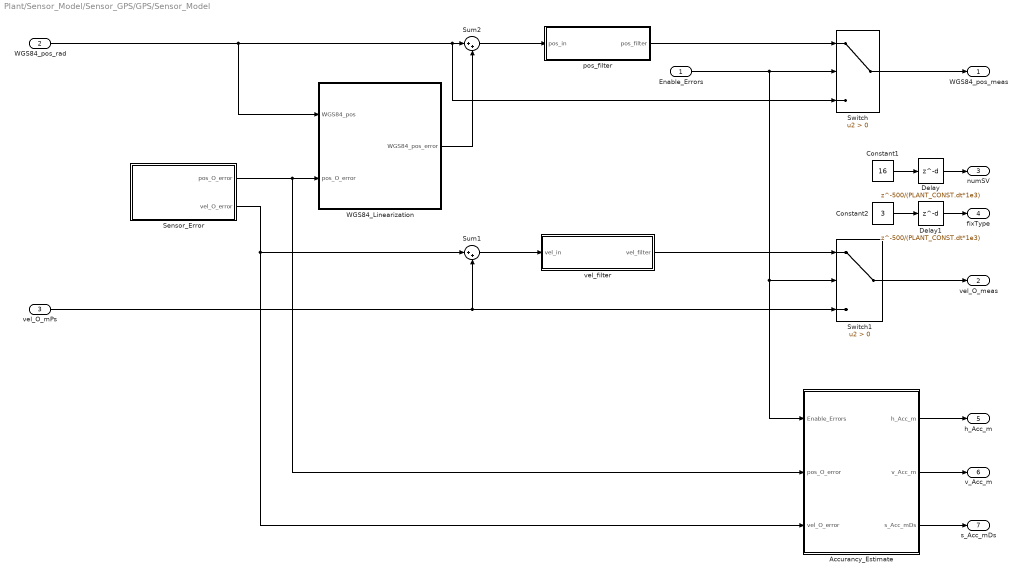
== system Plant/Sensor_Model/Sensor_GPS/GPS/Sensor_Model ==
  Enable_Errors : Inport
  WGS84_pos_rad : Inport  Port=2
  vel_O_mPs : Inport  Port=3
  Accurancy_Estimate : Subsystem
  Constant1 : Constant  Value=16  OutDataTypeStr=Inherit: Inherit via back propagation
  Constant2 : Constant  Value=3  OutDataTypeStr=Inherit: Inherit via back propagation
  Delay : Delay  DelayLength=500/(PLANT_CONST.dt*1e3)
  Delay1 : Delay  DelayLength=500/(PLANT_CONST.dt*1e3)
  Sensor_Error : Subsystem
  Sum1 : Sum  Inputs=|++
  Sum2 : Sum  Inputs=|++
  Switch : Switch  Criteria=u2 > Threshold
  Switch1 : Switch  Criteria=u2 > Threshold
  WGS84_Linearization : Subsystem
  pos_filter : Subsystem
  vel_filter : Subsystem
  WGS84_pos_meas : Outport
  vel_O_meas : Outport  Port=2
  numSV : Outport  Port=3
  fixType : Outport  Port=4
  h_Acc_m : Outport  Port=5
  v_Acc_m : Outport  Port=6
  s_Acc_mDs : Outport  Port=7
  wires:
  Constant2/1 -> Delay1/1
  Constant1/1 -> Delay/1
  Switch/1 -> WGS84_pos_meas/1
  Switch1/1 -> vel_O_meas/1
  Sum2/1 -> pos_filter/1(pos_in)
  Sensor_Error/1(pos_O_error) -> Accurancy_Estimate/2(pos_O_error), WGS84_Linearization/2(pos_O_error)
  Sum1/1 -> vel_filter/1(vel_in)
  Sensor_Error/2(vel_O_error) -> Accurancy_Estimate/3(vel_O_error), Sum1/1
  WGS84_Linearization/1(WGS84_pos_error) -> Sum2/2
  Accurancy_Estimate/1(h_Acc_m) -> h_Acc_m/1
  Accurancy_Estimate/3(s_Acc_mDs) -> s_Acc_mDs/1
  Accurancy_Estimate/2(v_Acc_m) -> v_Acc_m/1
  pos_filter/1(pos_filter) -> Switch/1
  WGS84_pos_rad/1 -> Switch/3, Sum2/1, WGS84_Linearization/1(WGS84_pos)
  vel_O_mPs/1 -> Switch1/3, Sum1/2
  vel_filter/1(vel_filter) -> Switch1/1
  Enable_Errors/1 -> Switch/2, Accurancy_Estimate/1(Enable_Errors), Switch1/2
  Delay/1 -> numSV/1
  Delay1/1 -> fixType/1

== system Plant/Sensor_Model/Sensor_IMU/Accelerometer/Bus_Constructor ==
  Output : Inport
  Bus Creator : BusCreator  Inputs=3
  Demux : Demux  Outputs=3
  Acc_Raw : Outport
  wires:
  Demux/2 -> Bus Creator/2  "Acc_y_mPs2"
  Demux/3 -> Bus Creator/3  "Acc_z_mPs2"
  Demux/1 -> Bus Creator/1  "Acc_x_mPs2"
  Bus Creator/1 -> Acc_Raw/1
  Output/1 -> Demux/1

== system Plant/Sensor_Model/Sensor_IMU/Accelerometer/Physical_Model ==
  States : Inport
  Enable_Errors : Inport  Port=2
  Sum : Sum  Inputs=|++
  Switch : Switch  Criteria=u2 > Threshold  OutDataTypeStr=single
  Vibration_Model : Subsystem  TreatAsAtomicUnit=on  mask{gain=Sensor_Model.Acc.Vibration.Gain}
      mask prompts: gain "Vibration gain"
      mask help: propeller vibration model
      settings: RTWSystemCode=Inline
  prop_vel : Subsystem
  specific_force : Subsystem
  sfor_B_mPs2 : Outport  Unit=m/s^2
  wires:
  States/1 -> specific_force/1(States), prop_vel/1(States)
  Switch/1 -> sfor_B_mPs2/1
  prop_vel/1(omega_radDs) -> Vibration_Model/1(prop_rot_radPs)
  specific_force/1(sfor_B_mPs2) -> Sum/2, Switch/3
  Enable_Errors/1 -> Switch/2
  Vibration_Model/1(vibration) -> Sum/1
  Sum/1 -> Switch/1

== system Plant/Sensor_Model/Sensor_IMU/Accelerometer/Sensor_Model ==
  Enable_Errors : Inport
  u : Inport  Port=2
  First Order LPF : FMT_Model_Lib/Filter/First Order LPF  fc=Sensor_Model.Acc.Cutoff_frequency_Hz
      settings: SourceProductName=FMT Toolbox
  Saturation : Saturate  UpperLimit=Sensor_Model.Acc.Upper_limit  LowerLimit=Sensor_Model.Acc.Lower_limit
  Sensor_Error : Subsystem
  Sensor_Noise : Subsystem
  Sum : Sum  Inputs=|++
  Switch : Switch  Criteria=u2 > Threshold
  y : Outport
  wires:
  Switch/1 -> y/1
  Saturation/1 -> Sum/1
  First Order LPF/1 -> Saturation/1
  Sensor_Error/1(y) -> First Order LPF/1
  Sensor_Noise/1(noise) -> Sum/2
  Enable_Errors/1 -> Switch/2
  u/1 -> Switch/3, Sensor_Error/1(u)
  Sum/1 -> Switch/1

== system Plant/Sensor_Model/Sensor_IMU/Gyroscope/Bus_Constructor ==
  Output : Inport
  Bus Creator : BusCreator  Inputs=3
  Demux : Demux  Outputs=3
  Gyro_Raw : Outport
  wires:
  Demux/1 -> Bus Creator/1  "Gyro_x_radPs"
  Demux/2 -> Bus Creator/2  "Gyro_y_radPs"
  Demux/3 -> Bus Creator/3  "Gyro_z_radPs"
  Bus Creator/1 -> Gyro_Raw/1
  Output/1 -> Demux/1

== system Plant/Sensor_Model/Sensor_IMU/Gyroscope/Physical_Model ==
  States : Inport
  Enable_Errors : Inport  Port=2
  Sum : Sum  Inputs=|++
  Switch : Switch  Criteria=u2 > Threshold
  Vibration_Model : Subsystem  TreatAsAtomicUnit=on  mask{gain=Sensor_Model.Gyro.Vibration.Gain}
      mask prompts: gain "Vibration gain"
      mask help: propeller vibration model
      settings: RTWSystemCode=Inline
  prop_vel : Subsystem
  rotation_speed : Subsystem
  gyr_B_radDs : Outport  Unit=rad/s
  wires:
  States/1 -> rotation_speed/1(States), prop_vel/1(States)
  Switch/1 -> gyr_B_radDs/1
  prop_vel/1(omega_radPs) -> Vibration_Model/1(prop_rot_radPs)
  rotation_speed/1(rot_radPs) -> Sum/2, Switch/3
  Enable_Errors/1 -> Switch/2
  Vibration_Model/1(vibration) -> Sum/1
  Sum/1 -> Switch/1

== system Plant/Sensor_Model/Sensor_IMU/Gyroscope/Sensor_Model ==
  Enable_Errors : Inport
  u : Inport  Port=2
  First Order LPF : FMT_Model_Lib/Filter/First Order LPF  fc=Sensor_Model.Gyro.Cutoff_frequency_Hz
      settings: SourceProductName=FMT Toolbox
  Saturation : Saturate  UpperLimit=Sensor_Model.Gyro.Range  LowerLimit=-Sensor_Model.Gyro.Range
  Sensor_Error : Subsystem
  Sensor_Noise : Subsystem
  Sum : Sum  Inputs=|++
  Switch : Switch  Criteria=u2 > Threshold
  y : Outport
  wires:
  Switch/1 -> y/1
  Saturation/1 -> Sum/1
  First Order LPF/1 -> Saturation/1
  Sensor_Error/1(y) -> First Order LPF/1
  Sensor_Noise/1(noise) -> Sum/2
  Enable_Errors/1 -> Switch/2
  u/1 -> Switch/3, Sensor_Error/1(u)
  Sum/1 -> Switch/1

== system Plant/Sensor_Model/Sensor_MAG/Magnetometer/Bus_Constructor ==
  Output : Inport
  Bus Creator : BusCreator  Inputs=3
  Demux : Demux  Outputs=3
  Mag_Raw : Outport
  wires:
  Demux/2 -> Bus Creator/2  "Mag_y_gauss"
  Demux/1 -> Bus Creator/1  "Mag_x_gauss"
  Bus Creator/1 -> Mag_Raw/1
  Demux/3 -> Bus Creator/3  "Mag_z_gauss"
  Output/1 -> Demux/1

== system Plant/Sensor_Model/Sensor_MAG/Magnetometer/Physical_Model ==
  States : Inport
  Bus Selector : BusSelector  OutputSignals=Plant_States.lat,Plant_States.lon
  Bus Selector1 : BusSelector  OutputSignals=Extended_States.M_BO
  Product : Product  Multiplication=Matrix(*)  RndMeth=Zero  InputSameDT=on  OutDataTypeStr=Inherit: Same as first input
  WMM_LUT : Subsystem  mask{wmm_magnitude=Sensor_Model.Mag.WMM_Mag, wmm_declination=Sensor_Model.Mag.WMM_Dec, wmm_inclination=Sensor_Model.Mag.WMM_Inc, resolution=10}
      mask prompts: wmm_magnitude "WMM Magnitude Lookup Table"; wmm_declination "WMM Declination Lookup Table"; wmm_inclination "WMM Inclination Lookup Table"; resolution "Resolution (deg)"
  magnetic_field : Subsystem
  mag_B_gauss : Outport  Unit=T  PortDimensions=[3 1]
  wires:
  States/1 -> Bus Selector1/1, Bus Selector/1
  Bus Selector/2 -> WMM_LUT/2(lon_rad)  "<lon>"
  Bus Selector/1 -> WMM_LUT/1(lat_rad)  "<lat>"
  Bus Selector1/1 -> Product/1  "<M_BO>"
  Product/1 -> mag_B_gauss/1
  magnetic_field/1(mag_O_gauss) -> Product/2
  WMM_LUT/1(magnitude_uT) -> magnetic_field/1(magnitude_uT)
  WMM_LUT/2(declination_deg) -> magnetic_field/2(declination_deg)
  WMM_LUT/3(inclination_deg) -> magnetic_field/3(inclination_deg)

== system Plant/Sensor_Model/Sensor_MAG/Magnetometer/Sensor_Model ==
  Enable_Errors : Inport
  u : Inport  Port=2
  Add : Sum  InputSameDT=on  OutDataTypeStr=Inherit: Same as first input
  Saturation : Saturate  UpperLimit=Sensor_Model.Mag.Upper_limit  LowerLimit=Sensor_Model.Mag.Lower_limit
  Sensor_Error : Subsystem
  Sensor_Noise : Subsystem
  Switch : Switch  Criteria=u2 > Threshold
  y : Outport
  wires:
  Switch/1 -> y/1
  Saturation/1 -> Add/1
  Sensor_Error/1(y) -> Saturation/1
  Sensor_Noise/1(noise) -> Add/2
  Enable_Errors/1 -> Switch/2
  u/1 -> Switch/3, Sensor_Error/1(u)
  Add/1 -> Switch/1

== system Plant/Actuators/Aerodynamics Forces and Moments/Aerodynamic Coefficients/Actuator increments/aileron ==
  alpha : Inport
  da : Inport  Port=2
  CD : Lookup2D  RowIndex=ada.dd  ColumnIndex=ada.alpha  Table=ada.CD
  CL : Constant  Value=0
  CL1 : Lookup2D  Commented=on  RowIndex=ada.dd  ColumnIndex=ada.alpha  Table=ada.CL
  CY : Lookup2D  RowIndex=ada.dd  ColumnIndex=ada.alpha  Table=ada.CY  LookUpMeth=Interpolation-Use End Values
  Cl : Lookup2D  RowIndex=ada.dd  ColumnIndex=ada.alpha  Table=ada.Cl
  Cm : Constant  Value=0
  Cm1 : Lookup2D  Commented=on  RowIndex=ada.dd  ColumnIndex=ada.alpha  Table=ada.Cm
  Cn : Lookup2D  RowIndex=ada.dd  ColumnIndex=ada.alpha  Table=ada.Cn
  Gain2 : Gain  Gain=-1
  Mux : Mux  Inputs=6
  Coeffs : Outport
  wires:
  Mux/1 -> Coeffs/1
  da/1 -> Gain2/1
  alpha/1 -> CY/2, Cl/2, Cn/2, CD/2
  CD/1 -> Mux/1
  CL/1 -> Mux/2
  Cm/1 -> Mux/5
  CY/1 -> Mux/3
  Cl/1 -> Mux/4
  Cn/1 -> Mux/6
  Gain2/1 -> CY/1, Cl/1, Cn/1, CD/1

== system Plant/Actuators/Aerodynamics Forces and Moments/Aerodynamic Coefficients/Actuator increments/elevator ==
  alpha : Inport
  de : Inport  Port=2
  CD : Lookup2D  RowIndex=ade.dd  ColumnIndex=ade.alpha  Table=ade.CD
  CL : Lookup2D  RowIndex=ade.dd  ColumnIndex=ade.alpha  Table=ade.CL
  CY : Constant  Value=0
  Cl : Constant  Value=0
  Cm : Lookup2D  RowIndex=ade.dd  ColumnIndex=ade.alpha  Table=ade.Cm
  Cn : Constant  Value=0
  Gain1 : Gain  Gain=-1
  Mux : Mux  Inputs=6
  Coeffs : Outport
  wires:
  de/1 -> Gain1/1
  alpha/1 -> Cm/2, CL/2, CD/2
  CL/1 -> Mux/2
  CD/1 -> Mux/1
  CY/1 -> Mux/3
  Cl/1 -> Mux/4
  Cn/1 -> Mux/6
  Cm/1 -> Mux/5
  Mux/1 -> Coeffs/1
  Gain1/1 -> Cm/1, CL/1, CD/1

== system Plant/Actuators/Aerodynamics Forces and Moments/Aerodynamic Coefficients/Actuator increments/rudder ==
  alpha : Inport
  dr : Inport  Port=2
  CD_dr : Lookup2D  RowIndex=adr.dd  ColumnIndex=adr.alpha  Table=adr.CD
  CL : Constant  Value=0
  CL_dr : Lookup2D  Commented=on  RowIndex=adr.dd  ColumnIndex=adr.alpha  Table=adr.CL
  CY_dr : Lookup2D  RowIndex=adr.dd  ColumnIndex=adr.alpha  Table=adr.CY
  Cl : Constant  Value=0
  Cl_dr : Lookup2D  Commented=on  RowIndex=adr.dd  ColumnIndex=adr.alpha  Table=adr.Cl
  Cm_dr : Lookup2D  RowIndex=adr.dd  ColumnIndex=adr.alpha  Table=adr.Cm  LookUpMeth=Interpolation-Use End Values
  Cn_dr : Lookup2D  RowIndex=adr.dd  ColumnIndex=adr.alpha  Table=adr.Cn
  Gain : Gain  Gain=-1
  Mux : Mux  Inputs=6
  Coeffs : Outport
  wires:
  Mux/1 -> Coeffs/1
  alpha/1 -> CY_dr/2, Cn_dr/2, CD_dr/2
  CL/1 -> Mux/2
  CD_dr/1 -> Mux/1
  CY_dr/1 -> Mux/3
  Cl/1 -> Mux/4
  Cm_dr/1 -> Mux/5
  Cn_dr/1 -> Mux/6
  dr/1 -> Gain/1
  Gain/1 -> CY_dr/1, Cm_dr/1, Cm_dr/2, Cn_dr/1, CD_dr/1

== system Plant/Actuators/Aerodynamics Forces and Moments/Aerodynamic Coefficients/body rate damping/p ==
  alpha : Inport
  CDp : Constant  Value=0
  CLp : Constant  Value=0
  CYp : Lookup  InputValues=adyn.alpha  Table=adyn.CYp
  Clp : Lookup  InputValues=adyn.alpha  Table=adyn.Clp
  Cmp : Constant  Value=0
  Cnp : Lookup  InputValues=adyn.alpha  Table=adyn.Cnp
  Mux : Mux  Inputs=6
  Coeffs : Outport
  wires:
  alpha/1 -> CYp/1, Clp/1, Cnp/1
  Cnp/1 -> Mux/6
  CYp/1 -> Mux/3
  Clp/1 -> Mux/4
  Mux/1 -> Coeffs/1
  CLp/1 -> Mux/2
  CDp/1 -> Mux/1
  Cmp/1 -> Mux/5

== system Plant/Actuators/Aerodynamics Forces and Moments/Aerodynamic Coefficients/body rate damping/q ==
  alpha : Inport
  CDq : Constant  Value=0
  CLq : Lookup  InputValues=adyn.alpha  Table=adyn.CLq
  CYq : Constant  Value=0
  Clq : Constant  Value=0
  Cmq : Lookup  InputValues=adyn.alpha  Table=adyn.Cmq
  Cnq : Constant  Value=0
  Mux : Mux  Inputs=6
  Coeffs : Outport
  wires:
  alpha/1 -> CLq/1, Cmq/1
  CLq/1 -> Mux/2
  Cmq/1 -> Mux/5
  CDq/1 -> Mux/1
  CYq/1 -> Mux/3
  Clq/1 -> Mux/4
  Cnq/1 -> Mux/6
  Mux/1 -> Coeffs/1

== system Plant/Actuators/Aerodynamics Forces and Moments/Aerodynamic Coefficients/body rate damping/r ==
  alpha : Inport
  CDr : Constant  Value=0
  CLr : Constant  Value=0
  CYr : Lookup  InputValues=adyn.alpha  Table=adyn.CYr
  Clr : Lookup  InputValues=adyn.alpha  Table=adyn.Clr
  Cmr : Constant  Value=0
  Cnr : Lookup  InputValues=adyn.alpha  Table=adyn.Cnr
  Mux : Mux  Inputs=6
  Coeffs : Outport
  wires:
  alpha/1 -> CYr/1, Clr/1, Cnr/1
  CYr/1 -> Mux/3
  Clr/1 -> Mux/4
  Cmr/1 -> Mux/5
  Cnr/1 -> Mux/6
  Mux/1 -> Coeffs/1
  CDr/1 -> Mux/1
  CLr/1 -> Mux/2

== system Plant/Sensor_Model/Sensor_Barometer/Barometer/Sensor_Model/Sensor_Error ==
  u : Inport
  Constant3 : Constant  Value=Sensor_Model.Baro.Bias  VectorParams1D=off  OutDataTypeStr=single
  Sum : Sum  Inputs=|++  InputSameDT=on  OutDataTypeStr=Inherit: Same as first input
  y : Outport
  wires:
  Sum/1 -> y/1
  u/1 -> Sum/1
  Constant3/1 -> Sum/2

== system Plant/Sensor_Model/Sensor_Barometer/Barometer/Sensor_Model/Sensor_Noise ==
  Random Source : dspsrcs4/Random Source  SrcType=Gaussian  NormMethod=Ziggurat  CltLength=12  MinVal=0  MaxVal=1  MeanVal=0  VarVal=Sensor_Model.Baro.Variance  RepMode=Repeatable  rawSeed=1  IsInherit=off  SampMode=Discrete  SampTime=-1  SampFrame=1  DataType=Single  OutComplex=Real  OutputFrames=off
  noise : Outport
  wires:
  Random Source/1 -> noise/1

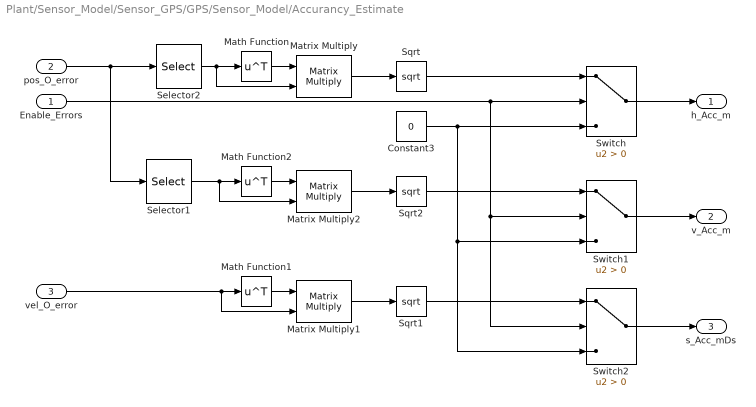
== system Plant/Sensor_Model/Sensor_GPS/GPS/Sensor_Model/Accurancy_Estimate ==
  Enable_Errors : Inport
  pos_O_error : Inport  Port=2
  vel_O_error : Inport  Port=3
  Constant3 : Constant  Value=0
  Math Function : Math  Operator=transpose  SaturateOnIntegerOverflow=on
  Math Function1 : Math  Operator=transpose  SaturateOnIntegerOverflow=on
  Math Function2 : Math  Operator=transpose  SaturateOnIntegerOverflow=on
  Matrix Multiply : Product  Multiplication=Matrix(*)
  Matrix Multiply1 : Product  Multiplication=Matrix(*)
  Matrix Multiply2 : Product  Multiplication=Matrix(*)
  Selector1 : Selector  InputPortWidth=3  IndexOptions=Index vector (dialog)  Indices=3  OutputSizes=1
  Selector2 : Selector  InputPortWidth=3  IndexOptions=Index vector (dialog)  Indices=[1 2]  OutputSizes=1
  Sqrt : Sqrt  OutputSignalType=real  SaturateOnIntegerOverflow=on
  Sqrt1 : Sqrt  OutputSignalType=real  SaturateOnIntegerOverflow=on
  Sqrt2 : Sqrt  OutputSignalType=real  SaturateOnIntegerOverflow=on
  Switch : Switch  Criteria=u2 > Threshold
  Switch1 : Switch  Criteria=u2 > Threshold
  Switch2 : Switch  Criteria=u2 > Threshold
  h_Acc_m : Outport
  v_Acc_m : Outport  Port=2
  s_Acc_mDs : Outport  Port=3
  wires:
  Switch/1 -> h_Acc_m/1
  pos_O_error/1 -> Selector1/1, Selector2/1
  Switch1/1 -> v_Acc_m/1
  Selector1/1 -> Math Function2/1, Matrix Multiply2/2
  Switch2/1 -> s_Acc_mDs/1
  Math Function1/1 -> Matrix Multiply1/1
  Math Function2/1 -> Matrix Multiply2/1
  Math Function/1 -> Matrix Multiply/1
  Selector2/1 -> Matrix Multiply/2, Math Function/1
  Matrix Multiply1/1 -> Sqrt1/1
  Matrix Multiply/1 -> Sqrt/1
  Matrix Multiply2/1 -> Sqrt2/1
  vel_O_error/1 -> Matrix Multiply1/2, Math Function1/1
  Sqrt/1 -> Switch/1
  Sqrt2/1 -> Switch1/1
  Enable_Errors/1 -> Switch2/2, Switch1/2, Switch/2
  Sqrt1/1 -> Switch2/1
  Constant3/1 -> Switch2/3, Switch1/3, Switch/3

== system Plant/Sensor_Model/Sensor_GPS/GPS/Sensor_Model/Sensor_Error ==
  Random Source : dspsrcs4/Random Source  SrcType=Gaussian  NormMethod=Ziggurat  CltLength=12  MinVal=0  MaxVal=1  MeanVal=0  VarVal=[0.2;0.2;0.4].^2  RepMode=Repeatable  rawSeed=1  IsInherit=off  SampMode=Discrete  SampTime=-1  SampFrame=1  DataType=Single  OutComplex=Real  OutputFrames=off
  Random Source1 : dspsrcs4/Random Source  SrcType=Gaussian  NormMethod=Ziggurat  CltLength=12  MinVal=0  MaxVal=1  MeanVal=0  VarVal=[0.01;0.01;0.01].^2  RepMode=Repeatable  rawSeed=1  IsInherit=off  SampMode=Discrete  SampTime=-1  SampFrame=1  DataType=Single  OutComplex=Real  OutputFrames=off
  pos_O_error : Outport
  vel_O_error : Outport  Port=2
  wires:
  Random Source/1 -> pos_O_error/1
  Random Source1/1 -> vel_O_error/1

== system Plant/Sensor_Model/Sensor_GPS/GPS/Sensor_Model/WGS84_Linearization ==
  WGS84_pos : Inport
  pos_O_error : Inport  Port=2
  Demux2 : Demux  Outputs=3
  Divide2 : Product  Inputs=/*
  LAT2FLAT Curve : FMT_Model_Lib/Transformation/LAT2FLAT Curve
      settings: SourceProductName=FMT Toolbox
  Terminator1 : Terminator
  Terminator2 : Terminator
  Vector Concatenate2 : Concatenate  NumInputs=3  Mode=Multidimensional array
  constant1 : Constant  Value=-1
  WGS84_pos_error : Outport
  wires:
  WGS84_pos/1 -> Demux2/1
  Demux2/1 -> LAT2FLAT Curve/1
  LAT2FLAT Curve/2 -> Vector Concatenate2/2
  pos_O_error/1 -> Divide2/2
  Vector Concatenate2/1 -> Divide2/1
  LAT2FLAT Curve/1 -> Vector Concatenate2/1
  Demux2/2 -> Terminator2/1
  Demux2/3 -> Terminator1/1
  constant1/1 -> Vector Concatenate2/3
  Divide2/1 -> WGS84_pos_error/1

== system Plant/Sensor_Model/Sensor_GPS/GPS/Sensor_Model/pos_filter ==
  pos_in : Inport
  Discrete FIR Filter : DiscreteFir
  pos_filter : Outport
  wires:
  Discrete FIR Filter/1 -> pos_filter/1
  pos_in/1 -> Discrete FIR Filter/1

== system Plant/Sensor_Model/Sensor_GPS/GPS/Sensor_Model/vel_filter ==
  vel_in : Inport
  Discrete FIR Filter : DiscreteFir
  vel_filter : Outport
  wires:
  Discrete FIR Filter/1 -> vel_filter/1
  vel_in/1 -> Discrete FIR Filter/1
